simulink model "TP1_DISTANCEMURS"  (R2024b)
settings: Solver=VariableStepAuto  StartTime=0.0  StopTime=100  RelTol=1e-3
values from neighbouring files (symbols this model uses):
  chemins_X_workspace = chemin_filtre(:, 1) * res    [planification_astar.m]    (also in planification_astar2.m = chemin_filtre(:, 1) * resolution)
  chemins_Y_workspace = chemin_filtre(:, 2) * res    [planification_astar.m]    (also in planification_astar2.m = chemin_filtre(:, 2) * resolution)
  murs = [murs ... (first row only)    [planification_astar.m]
libraries: slpidlib x4
settings Model: Creator=jdubuc222  LastModifiedBy=julien.dbc
settings OptimizationCC: ReuseModelBlockBuffer=off
settings RTWCC: GPUComputeCapability=3.5

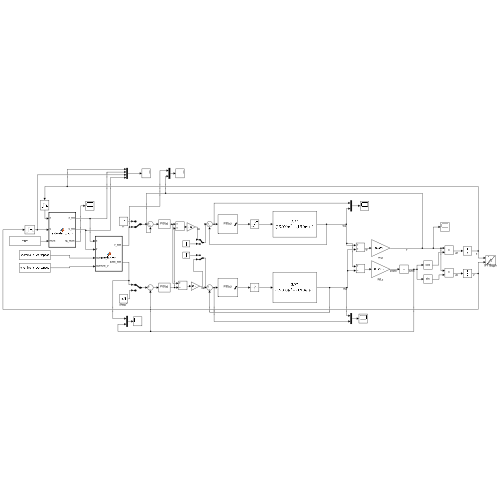
[thumbnail: Simulink's stored preview of the top-level diagram]
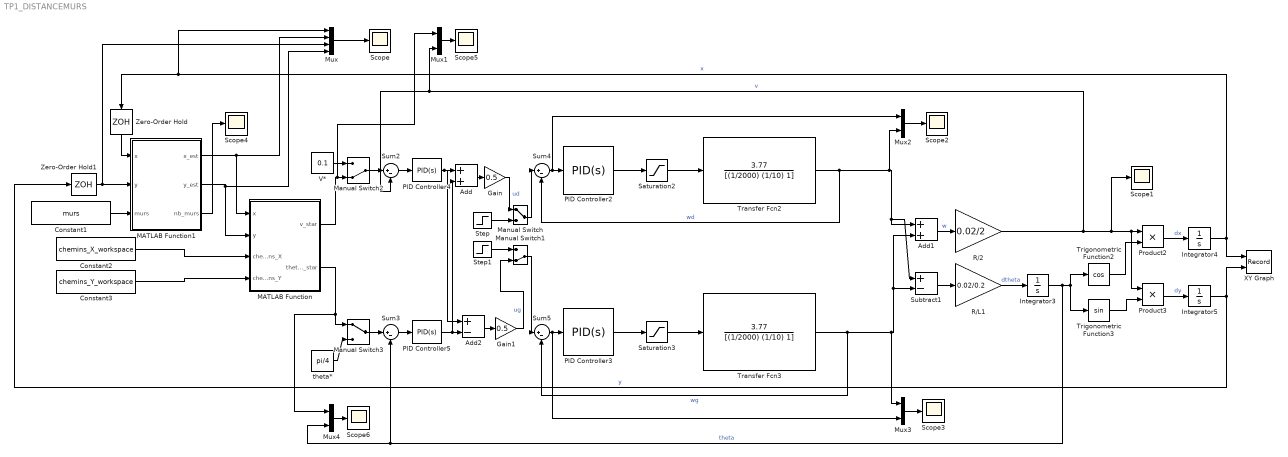
== system TP1_DISTANCEMURS ==
  Add : Sum
  Add1 : Sum
  Add2 : Sum  Inputs=+-
  Constant1 : Constant  Value=murs
  Constant2 : Constant  Value=chemins_X_workspace
  Constant3 : Constant  Value=chemins_Y_workspace
  Gain : Gain  Gain=0.5
  Gain1 : Gain  Gain=0.5
  Integrator3 : Integrator
  Integrator4 : Integrator  InitialCondition=chemins_X_workspace(1)
  Integrator5 : Integrator  InitialCondition=chemins_Y_workspace(1)
  MATLAB Function : MATLAB Function  TreatAsAtomicUnit=on
  MATLAB Function1 : MATLAB Function  TreatAsAtomicUnit=on
  Manual Switch : ManualSwitch
  Manual Switch1 : ManualSwitch  CurrentSetting=0
  Manual Switch2 : ManualSwitch  CurrentSetting=0
  Manual Switch3 : ManualSwitch
  Mux : Mux
  Mux{1..4} (4 alike) : Mux  Inputs=2
  PID Controller2 : slpidlib/PID Controller  Controller=PID  Form=Parallel  TimeDomain=Continuous-time  UseExternalTs=off  SampleTime=-1  IntegratorMethod=Forward Euler  FilterMethod=Forward Euler  ControllerParametersSource=internal  P=10  I=0  UseKiTs=off  D=0  UseExternalDerivativeSource=off  N=100  UseFilter=on  TunerSelectOption=Transfer Function Based (PID Tuner App)  InitialConditionSource=internal  InitialConditionForIntegrator=0  InitialConditionForFilter=0  DifferentiatorICPrevScaledInput=0  ExternalReset=none  TrackingMode=off  Kt=1  LimitOutput=on  SatLimitsSource=internal  UpperSaturationLimit=5  LowerSaturationLimit=-5  LinearizeAsGain=on  AntiWindupMode=clamping  Kb=1  LimitIntegrator=off  UpperIntegratorSaturationLimit=inf  LowerIntegratorSaturationLimit=-inf  POutMin=[]  POutMax=[]  IOutMin=[]  IOutMax=[]  DOutMin=[]  DOutMax=[]  NOutMin=[]  NOutMax=[]  SumOutMin=[]  SumOutMax=[]  SaturationOutMin=[]  SaturationOutMax=[]  PParamMin=[]  PParamMax=[]  IParamMin=[]  IParamMax=[]  DParamMin=[]  DParamMax=[]  NParamMin=[]  NParamMax=[]  KbParamMin=[]  KbParamMax=[]  KtParamMin=[]  KtParamMax=[]  KbOutMin=[]  KbOutMax=[]  KtOutMin=[]  KtOutMax=[]  IntegratorOutMin=[]  IntegratorOutMax=[]  FilterOutMin=[]  FilterOutMax=[]  SumI1OutMin=[]  SumI1OutMax=[]  SumI2OutMin=[]  SumI2OutMax=[]  SumI3OutMin=[]  SumI3OutMax=[]  SumI4OutMin=[]  SumI4OutMax=[]  SumDOutMin=[]  SumDOutMax=[]  DifferentiatorOutMin=[]  DifferentiatorOutMax=[]  FilterDiffOutCoefMin=[]  FilterDiffOutCoefMax=[]  ReciprocalOutMin=[]  ReciprocalOutMax=[]  SumDenOutMin=[]  SumDenOutMax=[]  SumNumOutMin=[]  SumNumOutMax=[]  DivideOutMin=[]  DivideOutMax=[]  UdiffTsProdOutMin=[]  UdiffTsProdOutMax=[]  NTsProdOutMin=[]  NTsProdOutMax=[]  UintegralTsProdOutMin=[]  UintegralTsProdOutMax=[]  UngainTsProdOutMin=[]  UngainTsProdOutMax=[]  ClampingZeroOutDataTypeStr=Inherit: Inherit via back propagation  ClampingZeroOutMin=[]  ClampingZeroOutMax=[]  FilterDenConstantOutDataTypeStr=Inherit: Inherit via back propagation  FilterDenConstantOutMin=[]  FilterDenConstantOutMax=[]  PCopyOutDataTypeStr=Inherit: Inherit via back propagation  PCopyOutMin=[]  PCopyOutMax=[]  NCopyOutDataTypeStr=Inherit: Inherit via back propagation  NCopyOutMin=[]  NCopyOutMax=[]  IntegratorContinuousStateAttributes=''  IntegratorStateMustResolveToSignalObject=off  IntegratorRTWStateStorageClass=Auto  FilterContinuousStateAttributes=''  FilterStateMustResolveToSignalObject=off  FilterRTWStateStorageClass=Auto  ParallelPVariant=InternalParameters  IdealPVariant=Disabled  IVariant=InternalParameters  DVariant=InternalParameters  IntegratorVariant=Continuous  SatVariant=Enabled  AWVariant=ContClampingParallel  PCopyVariant=Disabled  TRVariant=Disabled  FdbkBlocksVariant=Forward  IdealPFdbkVariant=Disabled  SatFdbkVariant=Disabled  DerivativeFilterVariant=ContFilter  NVariant=InternalParameters  NCopyVariant=Disabled  FilterICVariant=InternalICsFilter  IntegratorICVariant=InternalICs  ExternalResetVariant=Disabled  TRSumVariant=Passthrough  SumFdbkVariant=Disabled  SumVariant=Sum_PID  TsampFilterVariant=InternalTs  TsampNgainVariant=Passthrough  TsampIntegralVariant=Disabled_SignalSpec  ExternalSaturationOutDataTypeStr=Inherit: Same as second input  DerivativeSourceVariant=ErrorSignal  PreIntVariant=InternalPreInt
  PID Controller3 : slpidlib/PID Controller  Controller=PID  Form=Parallel  TimeDomain=Continuous-time  UseExternalTs=off  SampleTime=-1  IntegratorMethod=Forward Euler  FilterMethod=Forward Euler  ControllerParametersSource=internal  P=10  I=0  UseKiTs=off  D=0  UseExternalDerivativeSource=off  N=100  UseFilter=on  TunerSelectOption=Transfer Function Based (PID Tuner App)  InitialConditionSource=internal  InitialConditionForIntegrator=0  InitialConditionForFilter=0  DifferentiatorICPrevScaledInput=0  ExternalReset=none  TrackingMode=off  Kt=1  LimitOutput=on  SatLimitsSource=internal  UpperSaturationLimit=5  LowerSaturationLimit=-5  LinearizeAsGain=on  AntiWindupMode=clamping  Kb=1  LimitIntegrator=off  UpperIntegratorSaturationLimit=inf  LowerIntegratorSaturationLimit=-inf  POutMin=[]  POutMax=[]  IOutMin=[]  IOutMax=[]  DOutMin=[]  DOutMax=[]  NOutMin=[]  NOutMax=[]  SumOutMin=[]  SumOutMax=[]  SaturationOutMin=[]  SaturationOutMax=[]  PParamMin=[]  PParamMax=[]  IParamMin=[]  IParamMax=[]  DParamMin=[]  DParamMax=[]  NParamMin=[]  NParamMax=[]  KbParamMin=[]  KbParamMax=[]  KtParamMin=[]  KtParamMax=[]  KbOutMin=[]  KbOutMax=[]  KtOutMin=[]  KtOutMax=[]  IntegratorOutMin=[]  IntegratorOutMax=[]  FilterOutMin=[]  FilterOutMax=[]  SumI1OutMin=[]  SumI1OutMax=[]  SumI2OutMin=[]  SumI2OutMax=[]  SumI3OutMin=[]  SumI3OutMax=[]  SumI4OutMin=[]  SumI4OutMax=[]  SumDOutMin=[]  SumDOutMax=[]  DifferentiatorOutMin=[]  DifferentiatorOutMax=[]  FilterDiffOutCoefMin=[]  FilterDiffOutCoefMax=[]  ReciprocalOutMin=[]  ReciprocalOutMax=[]  SumDenOutMin=[]  SumDenOutMax=[]  SumNumOutMin=[]  SumNumOutMax=[]  DivideOutMin=[]  DivideOutMax=[]  UdiffTsProdOutMin=[]  UdiffTsProdOutMax=[]  NTsProdOutMin=[]  NTsProdOutMax=[]  UintegralTsProdOutMin=[]  UintegralTsProdOutMax=[]  UngainTsProdOutMin=[]  UngainTsProdOutMax=[]  ClampingZeroOutDataTypeStr=Inherit: Inherit via back propagation  ClampingZeroOutMin=[]  ClampingZeroOutMax=[]  FilterDenConstantOutDataTypeStr=Inherit: Inherit via back propagation  FilterDenConstantOutMin=[]  FilterDenConstantOutMax=[]  PCopyOutDataTypeStr=Inherit: Inherit via back propagation  PCopyOutMin=[]  PCopyOutMax=[]  NCopyOutDataTypeStr=Inherit: Inherit via back propagation  NCopyOutMin=[]  NCopyOutMax=[]  IntegratorContinuousStateAttributes=''  IntegratorStateMustResolveToSignalObject=off  IntegratorRTWStateStorageClass=Auto  FilterContinuousStateAttributes=''  FilterStateMustResolveToSignalObject=off  FilterRTWStateStorageClass=Auto  ParallelPVariant=InternalParameters  IdealPVariant=Disabled  IVariant=InternalParameters  DVariant=InternalParameters  IntegratorVariant=Continuous  SatVariant=Enabled  AWVariant=ContClampingParallel  PCopyVariant=Disabled  TRVariant=Disabled  FdbkBlocksVariant=Forward  IdealPFdbkVariant=Disabled  SatFdbkVariant=Disabled  DerivativeFilterVariant=ContFilter  NVariant=InternalParameters  NCopyVariant=Disabled  FilterICVariant=InternalICsFilter  IntegratorICVariant=InternalICs  ExternalResetVariant=Disabled  TRSumVariant=Passthrough  SumFdbkVariant=Disabled  SumVariant=Sum_PID  TsampFilterVariant=InternalTs  TsampNgainVariant=Passthrough  TsampIntegralVariant=Disabled_SignalSpec  ExternalSaturationOutDataTypeStr=Inherit: Same as second input  DerivativeSourceVariant=ErrorSignal  PreIntVariant=InternalPreInt
  PID Controller4 : slpidlib/PID Controller  Controller=PID  Form=Parallel  TimeDomain=Continuous-time  UseExternalTs=off  SampleTime=-1  IntegratorMethod=Forward Euler  FilterMethod=Forward Euler  ControllerParametersSource=internal  P=50  I=100  UseKiTs=off  D=0  UseExternalDerivativeSource=off  N=100  UseFilter=on  TunerSelectOption=Transfer Function Based (PID Tuner App)  InitialConditionSource=internal  InitialConditionForIntegrator=0  InitialConditionForFilter=0  DifferentiatorICPrevScaledInput=0  ExternalReset=none  TrackingMode=off  Kt=1  LimitOutput=off  SatLimitsSource=internal  UpperSaturationLimit=5  LowerSaturationLimit=-5  LinearizeAsGain=on  AntiWindupMode=clamping  Kb=1  LimitIntegrator=off  UpperIntegratorSaturationLimit=inf  LowerIntegratorSaturationLimit=-inf  POutMin=[]  POutMax=[]  IOutMin=[]  IOutMax=[]  DOutMin=[]  DOutMax=[]  NOutMin=[]  NOutMax=[]  SumOutMin=[]  SumOutMax=[]  SaturationOutMin=[]  SaturationOutMax=[]  PParamMin=[]  PParamMax=[]  IParamMin=[]  IParamMax=[]  DParamMin=[]  DParamMax=[]  NParamMin=[]  NParamMax=[]  KbParamMin=[]  KbParamMax=[]  KtParamMin=[]  KtParamMax=[]  KbOutMin=[]  KbOutMax=[]  KtOutMin=[]  KtOutMax=[]  IntegratorOutMin=[]  IntegratorOutMax=[]  FilterOutMin=[]  FilterOutMax=[]  SumI1OutMin=[]  SumI1OutMax=[]  SumI2OutMin=[]  SumI2OutMax=[]  SumI3OutMin=[]  SumI3OutMax=[]  SumI4OutMin=[]  SumI4OutMax=[]  SumDOutMin=[]  SumDOutMax=[]  DifferentiatorOutMin=[]  DifferentiatorOutMax=[]  FilterDiffOutCoefMin=[]  FilterDiffOutCoefMax=[]  ReciprocalOutMin=[]  ReciprocalOutMax=[]  SumDenOutMin=[]  SumDenOutMax=[]  SumNumOutMin=[]  SumNumOutMax=[]  DivideOutMin=[]  DivideOutMax=[]  UdiffTsProdOutMin=[]  UdiffTsProdOutMax=[]  NTsProdOutMin=[]  NTsProdOutMax=[]  UintegralTsProdOutMin=[]  UintegralTsProdOutMax=[]  UngainTsProdOutMin=[]  UngainTsProdOutMax=[]  ClampingZeroOutDataTypeStr=Inherit: Inherit via back propagation  ClampingZeroOutMin=[]  ClampingZeroOutMax=[]  FilterDenConstantOutDataTypeStr=Inherit: Inherit via back propagation  FilterDenConstantOutMin=[]  FilterDenConstantOutMax=[]  PCopyOutDataTypeStr=Inherit: Inherit via back propagation  PCopyOutMin=[]  PCopyOutMax=[]  NCopyOutDataTypeStr=Inherit: Inherit via back propagation  NCopyOutMin=[]  NCopyOutMax=[]  IntegratorContinuousStateAttributes=''  IntegratorStateMustResolveToSignalObject=off  IntegratorRTWStateStorageClass=Auto  FilterContinuousStateAttributes=''  FilterStateMustResolveToSignalObject=off  FilterRTWStateStorageClass=Auto  ParallelPVariant=InternalParameters  IdealPVariant=Disabled  IVariant=InternalParameters  DVariant=InternalParameters  IntegratorVariant=Continuous  SatVariant=Disabled  AWVariant=Passthrough  PCopyVariant=Disabled  TRVariant=Disabled  FdbkBlocksVariant=Forward  IdealPFdbkVariant=Disabled  SatFdbkVariant=Disabled  DerivativeFilterVariant=ContFilter  NVariant=InternalParameters  NCopyVariant=Disabled  FilterICVariant=InternalICsFilter  IntegratorICVariant=InternalICs  ExternalResetVariant=Disabled  TRSumVariant=Passthrough  SumFdbkVariant=Disabled  SumVariant=Sum_PID  TsampFilterVariant=InternalTs  TsampNgainVariant=Passthrough  TsampIntegralVariant=Disabled_SignalSpec  ExternalSaturationOutDataTypeStr=Inherit: Same as second input  DerivativeSourceVariant=ErrorSignal  PreIntVariant=InternalPreInt
  PID Controller5 : slpidlib/PID Controller  Controller=PID  Form=Parallel  TimeDomain=Continuous-time  UseExternalTs=off  SampleTime=-1  IntegratorMethod=Forward Euler  FilterMethod=Forward Euler  ControllerParametersSource=internal  P=14  I=0  UseKiTs=off  D=0  UseExternalDerivativeSource=off  N=100  UseFilter=on  TunerSelectOption=Transfer Function Based (PID Tuner App)  InitialConditionSource=internal  InitialConditionForIntegrator=0  InitialConditionForFilter=0  DifferentiatorICPrevScaledInput=0  ExternalReset=none  TrackingMode=off  Kt=1  LimitOutput=off  SatLimitsSource=internal  UpperSaturationLimit=5  LowerSaturationLimit=-5  LinearizeAsGain=on  AntiWindupMode=clamping  Kb=1  LimitIntegrator=off  UpperIntegratorSaturationLimit=inf  LowerIntegratorSaturationLimit=-inf  POutMin=[]  POutMax=[]  IOutMin=[]  IOutMax=[]  DOutMin=[]  DOutMax=[]  NOutMin=[]  NOutMax=[]  SumOutMin=[]  SumOutMax=[]  SaturationOutMin=[]  SaturationOutMax=[]  PParamMin=[]  PParamMax=[]  IParamMin=[]  IParamMax=[]  DParamMin=[]  DParamMax=[]  NParamMin=[]  NParamMax=[]  KbParamMin=[]  KbParamMax=[]  KtParamMin=[]  KtParamMax=[]  KbOutMin=[]  KbOutMax=[]  KtOutMin=[]  KtOutMax=[]  IntegratorOutMin=[]  IntegratorOutMax=[]  FilterOutMin=[]  FilterOutMax=[]  SumI1OutMin=[]  SumI1OutMax=[]  SumI2OutMin=[]  SumI2OutMax=[]  SumI3OutMin=[]  SumI3OutMax=[]  SumI4OutMin=[]  SumI4OutMax=[]  SumDOutMin=[]  SumDOutMax=[]  DifferentiatorOutMin=[]  DifferentiatorOutMax=[]  FilterDiffOutCoefMin=[]  FilterDiffOutCoefMax=[]  ReciprocalOutMin=[]  ReciprocalOutMax=[]  SumDenOutMin=[]  SumDenOutMax=[]  SumNumOutMin=[]  SumNumOutMax=[]  DivideOutMin=[]  DivideOutMax=[]  UdiffTsProdOutMin=[]  UdiffTsProdOutMax=[]  NTsProdOutMin=[]  NTsProdOutMax=[]  UintegralTsProdOutMin=[]  UintegralTsProdOutMax=[]  UngainTsProdOutMin=[]  UngainTsProdOutMax=[]  ClampingZeroOutDataTypeStr=Inherit: Inherit via back propagation  ClampingZeroOutMin=[]  ClampingZeroOutMax=[]  FilterDenConstantOutDataTypeStr=Inherit: Inherit via back propagation  FilterDenConstantOutMin=[]  FilterDenConstantOutMax=[]  PCopyOutDataTypeStr=Inherit: Inherit via back propagation  PCopyOutMin=[]  PCopyOutMax=[]  NCopyOutDataTypeStr=Inherit: Inherit via back propagation  NCopyOutMin=[]  NCopyOutMax=[]  IntegratorContinuousStateAttributes=''  IntegratorStateMustResolveToSignalObject=off  IntegratorRTWStateStorageClass=Auto  FilterContinuousStateAttributes=''  FilterStateMustResolveToSignalObject=off  FilterRTWStateStorageClass=Auto  ParallelPVariant=InternalParameters  IdealPVariant=Disabled  IVariant=InternalParameters  DVariant=InternalParameters  IntegratorVariant=Continuous  SatVariant=Disabled  AWVariant=Passthrough  PCopyVariant=Disabled  TRVariant=Disabled  FdbkBlocksVariant=Forward  IdealPFdbkVariant=Disabled  SatFdbkVariant=Disabled  DerivativeFilterVariant=ContFilter  NVariant=InternalParameters  NCopyVariant=Disabled  FilterICVariant=InternalICsFilter  IntegratorICVariant=InternalICs  ExternalResetVariant=Disabled  TRSumVariant=Passthrough  SumFdbkVariant=Disabled  SumVariant=Sum_PID  TsampFilterVariant=InternalTs  TsampNgainVariant=Passthrough  TsampIntegralVariant=Disabled_SignalSpec  ExternalSaturationOutDataTypeStr=Inherit: Same as second input  DerivativeSourceVariant=ErrorSignal  PreIntVariant=InternalPreInt
  Product2 : Product
  Product3 : Product
  R/2 : Gain  Gain=0.02/2
  R/L1 : Gain  Gain=0.02/0.2
  Saturation2 : Saturate  UpperLimit=5  LowerLimit=-5
  Saturation3 : Saturate  UpperLimit=5  LowerLimit=-5
  Scope{,1..6} (7 alike) : Scope
  Step : Step  After=6*pi  SampleTime=0
  Step1 : Step  After=6*pi  SampleTime=0
  Subtract1 : Sum  Inputs=+-
  Sum{2..5} (4 alike) : Sum  Inputs=|+-
  Transfer Fcn2 : TransferFcn  Numerator=[3.77]  Denominator=[(1/2000) (1/10) 1]
  Transfer Fcn3 : TransferFcn  Numerator=[3.77]  Denominator=[(1/2000) (1/10) 1]
  Trigonometric Function2 : Trigonometry  Operator=cos
  Trigonometric Function3 : Trigonometry
  V* : Constant  Value=0.1
  XY Graph : Record  FileSettingsInternal="{\"entries\":[{\"content\":{\"excelSettings\":{\"content\":{},\"type\":\"Streamout.ExcelSettings\"}},\"type\":\"Streamout.FileSettingStorage\",\"uuid\":\"\"}],\"packageUris\":[\"http:\\/\\/schema.mathworks.com\\/mf0\\/streamout_blocks\\/R2020a\"],\"version\":\"1.0\"}"  Layout=[1 1]  SignalsInternal="{\"entries\":[{\"content\":{\"signals\":[{\"content\":{\"blockPath\":[],\"dimensions\":[1],\"domain\":\"\",\"lineColor\":\"#a2142f\",\"plots\":[ 1 ],\"port\":1,\"sid\":[\"\"],\"signalID\":1,\"signalName\":\"x\"},\"type\":\"RecordBlkView.Signal\",\"uuid\":\"\"},{\"content\":{\"blockPath\":[],\"dimensions\":[1],\"domain\":\"\",\"lineColor\":\"#139fff\",\"plots\":[ 1 ],\"port\":2,\"sid\":[\"\"],\"signalID\":2,\"signalName\":\"y\"},\"type\":\"RecordBlkView.Signal\",\"uuid\":\"\"}]},\"type\":\"RecordBlkView.InputSignals\",\"uuid\":\"\"}],\"packageUris\":[\"http:\\/\\/schema.mathworks.com\\/mf0\\/streamout_blocks\\/R2020a\"],\"version\":\"1.0\"}"  VisualizationBindings="{\"xyplotplugin\":{\"info\":[{\"series\":[{\"bindingParametersList\":[{\"parameter\":\"X-Axis\",\"signalID\":1,\"signalName\":\"x\"},{\"parameter\":\"Y-Axis\",\"signalID\":2,\"signalName\":\"y\"}],\"seriesID\":0}],\"subplotID\":1}]}}"  CompatibilityTag=XY
  Zero-Order Hold : ZeroOrderHold  SampleTime=0.1
  Zero-Order Hold1 : ZeroOrderHold  SampleTime=0.1
  theta* : Constant  Value=pi/4
  wires:
  Manual Switch1/1 -> Sum5/1
  Sum5/1 -> Mux3/2, PID Controller3/1
  Gain/1 -> Manual Switch/1  "ud"
  Integrator5/1 -> Zero-Order Hold1/1, XY Graph/2  "y"
  Add/1 -> Gain/1
  Sum3/1 -> PID Controller5/1
  PID Controller3/1 -> Saturation3/1
  PID Controller4/1 -> Add2/1, Add/1
  Sum2/1 -> PID Controller4/1
  Step1/1 -> Manual Switch1/1
  Sum4/1 -> Mux2/1, PID Controller2/1
  Saturation2/1 -> Transfer Fcn2/1
  PID Controller5/1 -> Add2/2, Add/2
  Transfer Fcn3/1 -> Mux3/1, Subtract1/2, Add1/2, Sum5/2  "wg"
  Gain1/1 -> Manual Switch1/2  "ug"
  Mux3/1 -> Scope3/1
  Saturation3/1 -> Transfer Fcn3/1
  Add1/1 -> R/2/1  "w"
  Integrator3/1 -> Mux4/2, Sum3/2, Trigonometric Function3/1, Trigonometric Function2/1  "theta"
  Mux2/1 -> Scope2/1
  Step/1 -> Manual Switch/2
  Trigonometric Function3/1 -> Product3/2
  PID Controller2/1 -> Saturation2/1
  Add2/1 -> Gain1/1
  Product2/1 -> Integrator4/1  "dx"
  Integrator4/1 -> Mux/1, Zero-Order Hold/1, XY Graph/1  "x"
  Trigonometric Function2/1 -> Product2/2
  Manual Switch/1 -> Sum4/1
  Product3/1 -> Integrator5/1  "dy"
  Transfer Fcn2/1 -> Mux2/2, Subtract1/1, Add1/1, Sum4/2  "wd"
  R/2/1 -> Mux1/2, Sum2/2, Scope1/1, Product3/1, Product2/1  "v"
  Subtract1/1 -> R/L1/1
  R/L1/1 -> Integrator3/1  "dtheta"
  Manual Switch2/1 -> Sum2/1
  V*/1 -> Manual Switch2/1
  MATLAB Function/1(v_star) -> Mux1/1, Manual Switch2/2
  Manual Switch3/1 -> Sum3/1
  theta*/1 -> Manual Switch3/2
  MATLAB Function/2(theta_star) -> Mux4/1, Manual Switch3/1
  Constant3/1 -> MATLAB Function/4(chemins_Y)
  Constant2/1 -> MATLAB Function/3(chemins_X)
  Constant1/1 -> MATLAB Function1/3(murs)
  MATLAB Function1/1(x_est) -> Mux/2, MATLAB Function/1(x)
  MATLAB Function1/2(y_est) -> Mux/4, MATLAB Function/2(y)
  Zero-Order Hold/1 -> MATLAB Function1/1(x)
  Zero-Order Hold1/1 -> Mux/3, MATLAB Function1/2(y)
  Mux/1 -> Scope/1
  MATLAB Function1/3(nb_murs) -> Scope4/1
  Mux1/1 -> Scope5/1
  Mux4/1 -> Scope6/1

== matlab function TP1_DISTANCEMURS/MATLAB Function1 ==
  settings: updateMethod=DISCRETE
  data: x input; x_est output; y input; murs input; y_est output; nb_murs output
function [x_est, y_est, nb_murs] = estimateur_murs(x, y, murs)
% ESTIMATEUR_MURS  (code d'un bloc "MATLAB Function" dans Simulink)
%
% Ce bloc contient 2 choses :
%   1) un CAPTEUR VIRTUEL : à partir de la position vraie (x, y) il calcule
%      les distances aux murs, ajoute du bruit. La position vraie ne sert
%      QU'A fabriquer ces mesures.
%   2) un FILTRE DE KALMAN qui estime la position à partir des seules distances.
%
% Entrées : x, y    position vraie du robot (m), échantillonnée à DT (bloc Zero-Order Hold)
%           murs    matrice Nm x 4, une ligne par mur [ax ay bx by] (variable du workspace)
% Sorties : x_est, y_est   position estimée (m)
%           nb_murs        nombre de murs vus à cet instant

    DT     = 0.1;     % période d'échantillonnage : DOIT être la même que le Zero-Order Hold
    SIGMA  = 0.03;    % bruit de mesure de distance (m)
    PORTEE = 1.2;     % portée max du capteur (m)
    Q_ACC  = 0.05;    % "nervosité" supposée du robot (bruit d'accélération du modèle)

    Nm = size(murs, 1);

    % ---- Mémoire du filtre : état X = [x ; vx ; y ; vy] et incertitude Gam
    persistent X Gam
    if isempty(X)
        X   = [x + 0.4; 0; y - 0.4; 0];     % départ volontairement faux (40 cm), vitesse inconnue
        Gam = diag([1 0.1 1 0.1]);          % grande incertitude au départ
    end

    % ---- 1) CAPTEUR : distance signée à chaque mur : d = det(u, P - a)
    a  = murs(:, 1:2);
    b  = murs(:, 3:4);
    L  = sqrt(sum((b - a).^2, 2));
    u  = (b - a) ./ [L L];                          % vecteur unitaire le long du mur
    AP = [x - a(:,1),  y - a(:,2)];
    d  = u(:,1) .* AP(:,2) - u(:,2) .* AP(:,1);     % distance à la droite du mur
    t  = sum(AP .* u, 2);                           % position du pied de la perpendiculaire

    % mur visible : le pied tombe sur le segment, bon côté, dans la portée
    w = double((t >= 0) & (t <= L) & (d >= 0) & (d <= PORTEE));
    d_mes = d + SIGMA * randn(Nm, 1);               % mesure bruitée

    % ---- 2) KALMAN
    % prédiction (vitesse constante)
    A  = [1 DT 0 0;  0 1 0 0;  0 0 1 DT;  0 0 0 1];
    Qb = Q_ACC * [DT^3/3 DT^2/2;  DT^2/2 DT];
    G_alpha = [Qb zeros(2); zeros(2) Qb];
    X   = A * X;
    Gam = A * Gam * A' + G_alpha;

    % mesure rendue linéaire : y_i = d_i + u1*a2 - u2*a1 = -u2*x + u1*y
    % Les murs non vus ont une ligne de C nulle et un y nul : ils ne changent rien
    % (cela évite d'avoir un nombre de mesures variable dans Simulink).
    y_lin = w .* (d_mes + u(:,1) .* a(:,2) - u(:,2) .* a(:,1));
    C = [-w .* u(:,2),  zeros(Nm,1),  w .* u(:,1),  zeros(Nm,1)];

    % correction
    S   = C * Gam * C' + SIGMA^2 * eye(Nm);
    K   = Gam * C' / S;
    X   = X + K * (y_lin - C * X);
    Gam = Gam - K * C * Gam;
    Gam = (Gam + Gam') / 2;

    x_est   = X(1);
    y_est   = X(3);
    nb_murs = sum(w);
end

== matlab function TP1_DISTANCEMURS/MATLAB Function ==
  settings: updateMethod=DISCRETE
  data: x input; v_star output; y input; chemins_X input; chemins_Y input; theta_star output
function [v_star, theta_star] = planificateur(x, y, chemins_X, chemins_Y)
% PLANIFICATEUR  (code du bloc "MATLAB Function" dans Simulink)
%
% Entrées  : x, y               position du robot (m)
%            chemins_X/Y        liste des waypoints A* (m)
% Sorties  : v_star             consigne de vitesse (m/s)
%            theta_star         consigne de cap (rad)
%
% Principe : le robot vise le waypoint courant. Quand il est à moins de
% SEUIL du waypoint, il passe au suivant. Après le dernier, il s'arrête
% en gardant son dernier cap (sinon theta_star retomberait à 0 et le
% robot ferait demi-tour sur place).

    SEUIL = 0.10;    % distance (m) à laquelle un waypoint est "atteint"
    KV    = 0.5;     % gain : vitesse proportionnelle à la distance restante
    VMAX  = 0.3;     % vitesse max (m/s)

    % Mémoire entre deux pas de simulation
    persistent k_cible cap fini
    if isempty(k_cible)
        k_cible = 1;       % index du waypoint visé
        cap     = 0;       % dernier cap calculé
        fini    = false;   % true quand le dernier waypoint est atteint
    end

    % 1) Waypoint atteint ? -> on passe au suivant (ou on termine)
    if ~fini
        d = hypot(chemins_X(k_cible) - x, chemins_Y(k_cible) - y);
        if d < SEUIL
            if k_cible < numel(chemins_X)
                k_cible = k_cible + 1;
            else
                fini = true;
            end
        end
    end

    % 2) Fin du trajet : vitesse nulle, cap conservé
    if fini
        v_star     = 0;
        theta_star = cap;
        return;
    end

    % 3) Sinon : on vise le waypoint courant
    xB = chemins_X(k_cible);
    yB = chemins_Y(k_cible);
    d  = hypot(xB - x, yB - y);

    v_star     = min(KV * d, VMAX);        % ralentit à l'approche, plafonné à VMAX
    cap        = atan2(yB - y, xB - x);    % direction du waypoint
    theta_star = cap;
end
